simulink model "STSDiagram"  (R2025a)
settings: Solver=VariableStepAuto  StartTime=0.0  StopTime=5  RelTol=1e-3
libraries: spsThyristorLib x6, spsCurrentMeasurementLib x3, spsParallelRLCLoadLib x3, spsVoltageMeasurementLib x3, spsThreePhaseSourceLib x1, sps_lib x1
settings Model: Creator=Ayush  LastModifiedBy=Ayush

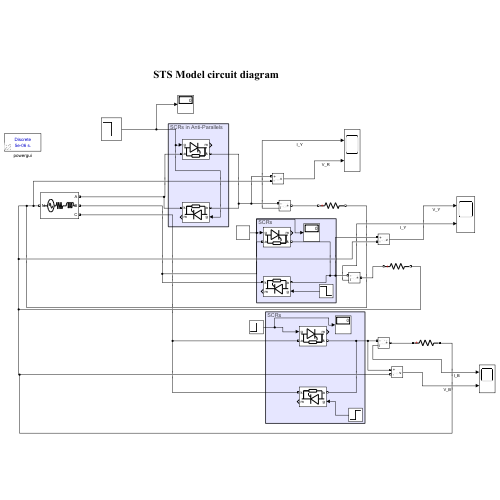
[thumbnail: Simulink's stored preview of the top-level diagram]
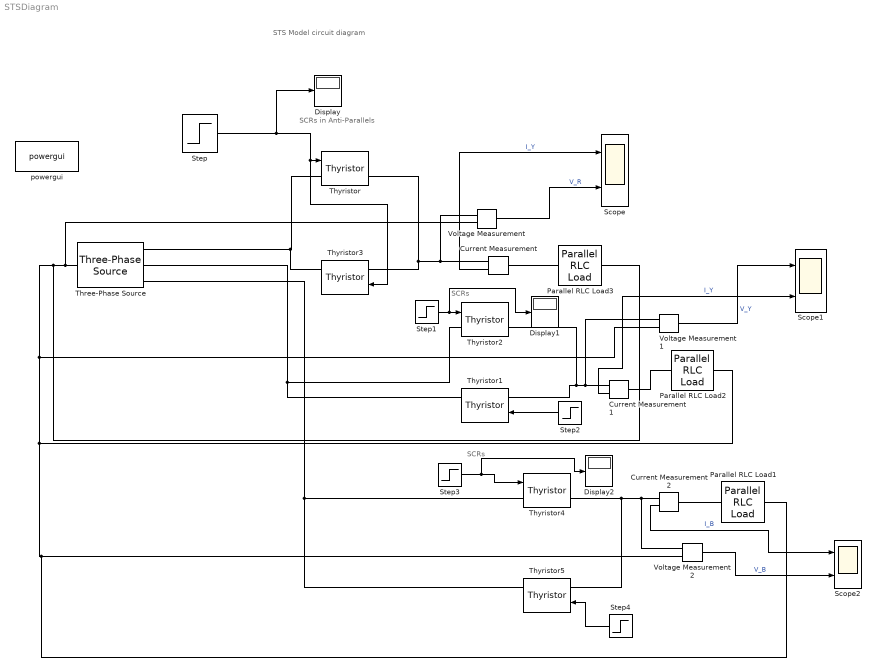
== system STSDiagram ==
  note: STS Model circuit diagram
  note: SCRs
  note: SCRs
  note: SCRs in Anti-Parallels
  Current Measurement : spsCurrentMeasurementLib/Current Measurement  PhasorSimulation=off  OutputType=Complex  PSBequivalent=0
  Current Measurement1 : spsCurrentMeasurementLib/Current Measurement  PhasorSimulation=off  OutputType=Complex  PSBequivalent=0
  Current Measurement2 : spsCurrentMeasurementLib/Current Measurement  PhasorSimulation=off  OutputType=Complex  PSBequivalent=0
  Display : Display
  Display1 : Display
  Display2 : Display
  Parallel RLC Load1 : spsParallelRLCLoadLib/Parallel RLC Load  LConnTagsString=a  RConnTagsString=__new0  NominalVoltage=239.6  NominalFrequency=50  ActivePower=12e3  InductivePower=0  CapacitivePower=0  Setx0=off  InitialVoltage=0  SetiL0=off  InitialCurrent=0  Measurements=None  LoadType=constant Z
      settings: AttributesFormatString=\n  LibrarySourceBlock=sps_lib/Passives/Parallel RLC Load
  Parallel RLC Load2 : spsParallelRLCLoadLib/Parallel RLC Load  LConnTagsString=a  RConnTagsString=__new0  NominalVoltage=239.6  NominalFrequency=50  ActivePower=10e3  InductivePower=0  CapacitivePower=0  Setx0=off  InitialVoltage=0  SetiL0=off  InitialCurrent=0  Measurements=None  LoadType=constant Z
      settings: AttributesFormatString=\n  LibrarySourceBlock=sps_lib/Passives/Parallel RLC Load
  Parallel RLC Load3 : spsParallelRLCLoadLib/Parallel RLC Load  LConnTagsString=a  RConnTagsString=__new0  NominalVoltage=239.6  NominalFrequency=50  ActivePower=5e3  InductivePower=0  CapacitivePower=0  Setx0=off  InitialVoltage=0  SetiL0=off  InitialCurrent=0  Measurements=None  LoadType=constant Z
      settings: AttributesFormatString=\n  LibrarySourceBlock=sps_lib/Passives/Parallel RLC Load
  Scope : Scope  NumInputPorts=2
      settings: ActiveDisplayYMinimum=-137.56335918636114  ActiveDisplayYMaximum=513.54198839543915
  Scope1 : Scope  NumInputPorts=2
      settings: ActiveDisplayYMinimum=-260.16434390326197  ActiveDisplayYMaximum=401.86162416436997
  Scope2 : Scope  NumInputPorts=2
      settings: ActiveDisplayYMinimum=-1213.8720829842719  ActiveDisplayYMaximum=1117.8205542822734  DataLoggingVariableName=ScopeData2
  Step : Step  Time=2  Before=1  After=0  SampleTime=0
  Step1 : Step  Time=3  Before=1  After=0  SampleTime=0
  Step2 : Step  Time=3  Before=1  After=0  SampleTime=0
  Step3 : Step  Time=4  SampleTime=0
  Step4 : Step  Time=4  SampleTime=0
  Three-Phase Source : spsThreePhaseSourceLib/Three-Phase Source  InternalConnection=Yn  VoltagePhases=off  Voltage=415  PhaseAngle=0  Voltage_phases=[25e3 25e3 25e3]/sqrt(3)  PhaseAngles_phases=[0 -120 +120]  Frequency=50  NonIdealSource=on  SpecifyImpedance=on  Resistance=0.8929  Inductance=16.58e-3  ShortCircuitLevel=100e6  BaseVoltage=415  XRratio=7  BusType=swing  Pref=10e3  Qref=0  Prefabc=[10e3, 10e3, 10e3]  Qrefabc=[0, 0, 0]  Qmin=-inf  Qmax=inf
  Thyristor{,1..5} (6 alike) : spsThyristorLib/Thyristor  Ron=0.001  Lon=0  Vf=0.8  IC=0  Rs=500  Cs=250e-9  Measurements=on
  Voltage Measurement : spsVoltageMeasurementLib/Voltage Measurement  PhasorSimulation=off  OutputType=Complex  PSBequivalent=0
  Voltage Measurement1 : spsVoltageMeasurementLib/Voltage Measurement  PhasorSimulation=off  OutputType=Complex  PSBequivalent=0
  Voltage Measurement2 : spsVoltageMeasurementLib/Voltage Measurement  PhasorSimulation=off  OutputType=Complex  PSBequivalent=0
  powergui : sps_lib/powergui  Priority=1  SimulationMode=Discrete  SampleTime=5e-6  frequency=60  Iterations=50  frequencyindice=50  Pbase=100e6  ErrMax=1e-4  UnitsV=kV  UnitsW=MW  buscounter=0  FunctionMessages=off  echomessages=off  EnableUseOfTLC=off  CurrentSourceSwitches=off  DisableSnubberDevices=off  DisableRonSwitches=off  DisableVfSwitches=off  DisplayEquations=off  AutomaticDiscreteSolvers=off  SolverType=Tustin/Backward Euler (TBE)  Interpol=off  ExternalGateDelay=off  methode=off  Ts=100  x0status=blocks  SPID=on  SwTol=0  HookPort=off  NonlinearTolerance=1e-4  nMaxIteration=100  ContinueOnMaxIteration=off  RestoreLinks=warning  ResistiveCurrentMeasurement=off  Frange=[0:2:500]  Ylog=off  Xlog=on  ShowGrid=off  save=off  variable=ZData  structure=0  ZoomFFT=off  StartTime=0.0  cycles=1  DisplayStyle=1  fundamental=60  FreqAxis=off  MaxFrequency=1000  frequencyindicesteady=1  RmsSteady=1  display=off
  wires:
  Step/1 -> Display/1, Thyristor/1, Thyristor3/1
  Voltage Measurement/1 -> Scope/2  "V_R"
  Current Measurement/1 -> Scope/1  "I_Y"
  Step1/1 -> Display1/1, Thyristor2/1
  Step2/1 -> Thyristor1/1
  Step4/1 -> Thyristor5/1
  Step3/1 -> Display2/1, Thyristor4/1
  Voltage Measurement1/1 -> Scope1/1  "V_Y"
  Current Measurement1/1 -> Scope1/2  "I_Y"
  Current Measurement2/1 -> Scope2/1  "I_B"
  Voltage Measurement2/1 -> Scope2/2  "V_B"
  connections:
  Thyristor3/LConn1 -- Thyristor/RConn1 -- Voltage Measurement/LConn1 -- Current Measurement/RConn1
  Parallel RLC Load1/RConn1 -- Voltage Measurement2/LConn2 -- Parallel RLC Load2/RConn1 -- Voltage Measurement1/LConn2 -- Parallel RLC Load3/RConn1 -- Voltage Measurement/LConn2 -- Three-Phase Source/LConn1
  Voltage Measurement2/LConn1 -- Current Measurement2/RConn1 -- Thyristor5/LConn1 -- Thyristor4/RConn1
  Parallel RLC Load2/LConn1 -- Current Measurement1/LConn1
  Thyristor1/RConn1 -- Three-Phase Source/RConn2 -- Thyristor2/LConn1
  Parallel RLC Load1/LConn1 -- Current Measurement2/LConn1
  Thyristor/LConn1 -- Thyristor3/RConn1 -- Three-Phase Source/RConn1
  Current Measurement1/RConn1 -- Thyristor1/LConn1 -- Thyristor2/RConn1 -- Voltage Measurement1/LConn1
  Thyristor5/RConn1 -- Three-Phase Source/RConn3 -- Thyristor4/LConn1
  Parallel RLC Load3/LConn1 -- Current Measurement/LConn1
